simulink model "BLDC_simulator"  (R2024a)
settings: Solver=ode4  StartTime=0.0  StopTime=T  MaxStep=20e-5  RelTol=1e-3  EnableMultiTasking=on
PreLoadFcn:
  | % load scdfocmotorPIDTuning_initial
  | % set_parameters
values from neighbouring files (symbols this model uses):
  current_loop = 1    [BLDC_simulator_init_control.m]    (also in BLDC_simulator_init_control_net_v2_stats_multi.m)
  i_omega = 2.497  * coeff(rand())    [set_parameters_perturbed.m]
  paramPwmCompareAtZeroVolt = 330    [set_parameters_perturbed.m]
  paramPwmCompareMax = 660    [set_parameters_perturbed.m]
  paramPwmComparePerVolt = paramPwmCompareMax/2/BLDC.RatedVoltage    [set_parameters_perturbed.m]
  speed_loop = 1    [BLDC_simulator_init_control.m]    (also in BLDC_simulator_init_control_net_v2_stats_multi.m)
undefined symbols (not defined in the file or in its folder): BLDC, inverter, PID_current, PID_speed, pwm, sampleTime
libraries: nesl_utility x13, fl_lib x12, ee_lib x8, slpidlib x3, simulink x1
(part 1 of 2)
settings Model: ExtModeTrigDuration=8  Creator=The MathWorks, Inc.  LastModifiedBy=39340
settings SolverCC: ZeroCrossAlgorithm=Adaptive  AlgebraicLoopSolver=TrustRegion  MaxZcPerStep=1
settings DataIOCC: InitialState=getstatestruct(op_speedloop)  LimitDataPoints=on  SaveFormat=Structure  InspectSignalLogs=on
settings OptimizationCC: ReuseModelBlockBuffer=off  LifeSpan=Inf
settings DebuggingCC: SolverPrmCheckMsg=warning  InheritedTsInSrcMsg=none  ParameterPrecisionLossMsg=none  UnconnectedInputMsg=warning  UnconnectedOutputMsg=warning  UnconnectedLineMsg=warning  AllowSymbolicDim=off  SFUnexpectedBacktrackingDiag=warning  SFNoUnconditionalDefaultTransitionDiag=warning  SFExecutionAtInitializationDiag=none  ArithmeticOperatorsInVariantConditions=warning
settings HardwareCC: ProdBitPerPointer=32  ProdBitPerSizeT=32  ProdBitPerPtrDiffT=32  ProdLargestAtomicFloat=None  ProdIntDivRoundTo=Undefined  ProdEndianess=Unspecified  ProdWordSize=32  ProdHWDeviceType=ASIC/FPGA->ASIC/FPGA  ProdEqTarget=off
settings ModelReferenceCC: EnableRefExpFcnMdlSchedulingChecks=on  PropagateSignalLabelsOutOfModel=off
settings SFSimCC: SimUseLocalCustomCode=off  CustomCodeUndefinedFunction=UseInterfaceOnly
settings RTWCC: RTWUseLocalCustomCode=off  GPUComputeCapability=3.5  DLArmComputeVersion=19.05
settings CodeAppCC: StateflowObjectComments=on
settings GRTTargetCC: TargetLangStandard=C89/C90 (ANSI)
settings ConfigComp: CovMetricSettings=dw  CovSaveCumulativeToWorkspaceVar=on  CovSaveSingleToWorkspaceVar=on  CovExternalEMLEnable=off  CovSFcnEnable=off
settings SimscapeCC: SimscapeNormalizeSystem=off  SimscapeOperatingPoint=op_innerloop

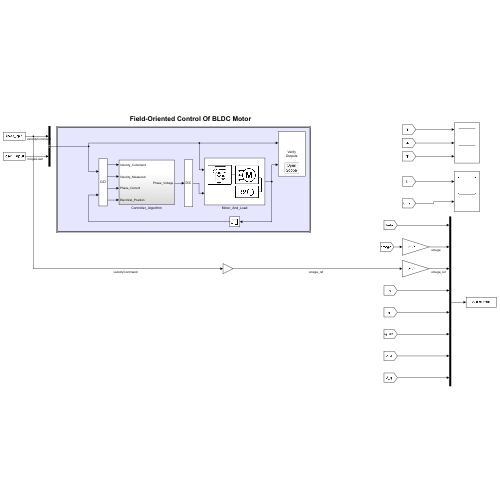
[thumbnail: Simulink's stored preview of the top-level diagram]
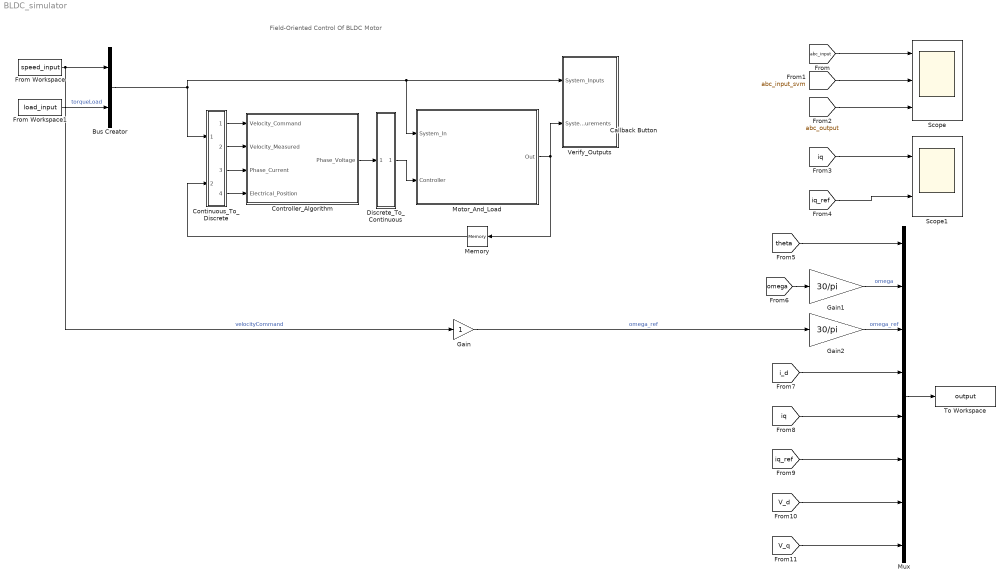
== system BLDC_simulator ==
  note: Field-Oriented Control Of BLDC Motor
  Bus Creator : BusCreator  Inputs=2
  Callback Button : CustomCallbackButton  Configuration="{\"components\":[{\"name\":\"BackgroundImageComponent\",\"settings\":{\"image\":{\"size\":[0,0],\"src\":\"default\",\"srcOrientation\":\"Right\"},\"position\":[0,0,1,1]}},{\"name\":\"ButtonStateComponent\",\"settings\":{\"buttonType\":\"momentary\",\"clickFcn\":\"open_system([bdroot, '\\/Verify_Outputs\\/System_Response']);\\n\",\"onValue\":1,\"position\":[0,0,1,1],\"pressDelay\":\"500\",\"pressFcn\":\"\",\"repeatInterval\":\"0\",\"states\":[{\"horizontalAlignment\":\"center\",\"image\":{\"position\":[0,0,1,1],\"src\":\"default\",\"srcOrientation\":\"Right\"},\"label\":{\"color\":[0.01176470588,0.01176470588,0.01176470588,1],\"icon\":{\"size\":[0,0],\"src\":\"default\",\"srcOrientation\":\"Right\"},\"iconPlacement\":\"left\",\"text\":{\"content\":\"Open Scope\"}},\"labelOffset\":[0,0],\"verticalAlignment\":\"middle\"},{\"horizontalAlignment\":\"center\",\"image\":{\"position\":[0,0,1,1],\"src\":\"default\",\"srcOrientation\":\"Right\"},\"label\":{\"color\":[0.01176470588,0.01176470588,0.01176470588,1],\"icon\":{\"size\":[0,0],\"src\":\"default\",\"srcOrientation\":\"Right\"},\"iconPlacement\":\"left\",\"text\":{\"content\":\"Open Scope\"}},\"labelOffset\":[0,0],\"verticalAlignment\":\"middle\"},{\"horizontalAlignment\":\"center\",\"image\":{\"position\":[0,0,1,1],\"src\":\"default\",\"srcOrientation\":\"Right\"},\"label\":{\"color\":[0.01176470588,0.01176470588,0.01176470588,1],\"icon\":{\"size\":[0,0],\"src\":\"default\",\"srcOrientation\":\"Right\"},\"iconPlacement\":\"left\",\"text\":{\"content\":\"Open Scope\"}},\"labelOffset\":[0,0],\"verticalAlignment\":\"middle\"},{\"horizontalAlignment\":\"center\",\"image\":{\"position\":[0,0,1,1],\"src\":\"default\",\"srcOrientation\":\"Right\"},\"label\":{\"color\":[0.01176470588,0.01176470588,0.01176470588,1],\"icon\":{\"size\":[0,0],\"src\":\"default\",\"srcOrientation\":\"Right\"},\"iconPlacement\":\"left\",\"text\":{\"content\":\"Open Scope\"}},\"labelOffset\":[0,0],\"verticalAlignment\":\"middle\"}]}},{\"name\":\"ForegroundImageComponent\",\"settings\":{\"image\":{\"size\":[0,0],\"src\":\"default\",\"srcOrientation\":\"Right\"},\"isForeground\":1,\"position\":[0,0,1,1]}}],\"settings\":{\"BindingType\":\"standalone\",\"backgroundColor\":[244,244,244,1],\"backgroundOffset\":0.2,\"backgroundOpacity\":1,\"fixedAspectRatio\":\"off\",\"foregroundColor\":[0.01176470588,0.01176470588,0.01176470588,1],\"migratedFromLegacy\":true,\"useBackgroundColor\":true,\"variant\":\"callback\",\"version\":\"R2023a\"},\"type\":\"Button\"}"  CustomBackgroundColor="{\"color\":[0.9568627451,0.9568627451,0.9568627451],\"show\":true}"
  Continuous_To_Discrete : Subsystem
      mask Display: fprintf('C/D')
  Controller_Algorithm : Subsystem
  Discrete_To_Continuous : Subsystem  Description=""
      mask Display: fprintf('D/C')
  From Workspace : FromWorkspace  VariableName=speed_input  SampleTime=-1  OutputAfterFinalValue=Holding final value
  From Workspace1 : FromWorkspace  VariableName=load_input  SampleTime=-1  OutputAfterFinalValue=Holding final value
  Gain : Gain
  Gain1 : Gain  Gain=30/pi
  Gain2 : Gain  Gain=30/pi
  Memory : Memory
  Motor_And_Load : Subsystem
      mask Display: image('focVelocityMotorAndLoadMask.png')
  Mux : Mux  Inputs=8
  Scope : Scope  NumInputPorts=3
  Scope1 : Scope  NumInputPorts=2
  To Workspace : ToWorkspace  VariableName=output  SaveFormat=Structure With Time  SampleTime=-1
      settings: Decimation=1e-2/sampleTime.CurrentControl
  Verify_Outputs : Subsystem  Description=|
      | System Analysis for Speed Control Design
      | 
      | Analyize and plot signals used to analyize performance of
      | speed  control designs
      mask Display: fprintf('Verify\nOutputs')
  wires:
  Discrete_To_Continuous/1(Motor_Commands) -> Motor_And_Load/2(Controller)
  Motor_And_Load/1(Out) -> Memory/1, Verify_Outputs/2(System_Measurements)
  Bus Creator/1 -> Continuous_To_Discrete/1(System_Inputs), Verify_Outputs/1(System_Inputs), Motor_And_Load/1(System_In)
  Continuous_To_Discrete/1(Velocity_Command) -> Controller_Algorithm/1(Velocity_Command)
  Controller_Algorithm/1(Phase_Voltage) -> Discrete_To_Continuous/1(Phase_Voltages)
  Continuous_To_Discrete/3(Phase_Currents) -> Controller_Algorithm/3(Phase_Current)
  Continuous_To_Discrete/4(Electrical_Position) -> Controller_Algorithm/4(Electrical_Position)
  Continuous_To_Discrete/2(Velocity_Measured) -> Controller_Algorithm/2(Velocity_Measured)
  Memory/1 -> Continuous_To_Discrete/2(Motor_Measurements)
  [abc_input] -> Scope/1
  [abc_input_svm] -> Scope/2
  [abc_output] -> Scope/3
  [iq] -> Scope1/1
  [iq_ref] -> Scope1/2
  From Workspace/1 -> Gain/1, Bus Creator/1  "velocityCommand"
  From Workspace1/1 -> Bus Creator/2  "torqueLoad"
  [theta] -> Mux/1
  [omega] -> Gain1/1
  Gain/1 -> Gain2/1  "omega_ref"
  [i_d] -> Mux/4
  [iq] -> Mux/5
  [iq_ref] -> Mux/6
  [V_d] -> Mux/7
  [V_q] -> Mux/8
  Mux/1 -> To Workspace/1
  Gain1/1 -> Mux/2  "omega"
  Gain2/1 -> Mux/3  "omega_ref"

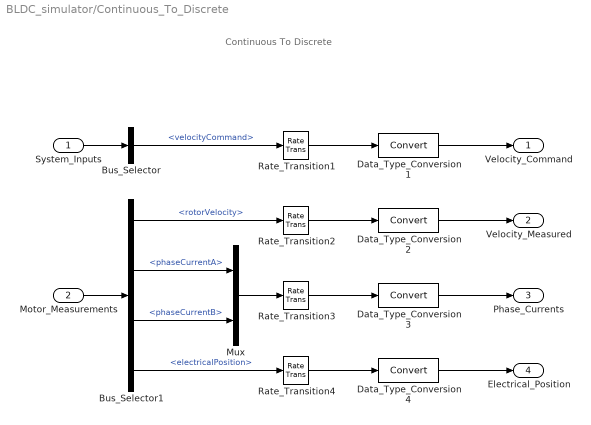
== system BLDC_simulator/Continuous_To_Discrete ==
  note: Continuous To Discrete
  System_Inputs : Inport
  Motor_Measurements : Inport  Port=2
  Bus_Selector : BusSelector  OutputSignals=velocityCommand
  Bus_Selector1 : BusSelector  OutputSignals=motor.rotorVelocity,motor.phaseCurrentA,motor.phaseCurrentB,motor.electricalPosition
  Data_Type_Conversion{1..4} (4 alike) : DataTypeConversion  SaturateOnIntegerOverflow=off  RndMeth=Floor
  Mux : Mux  Inputs=2
  Rate_Transition{1..4} (4 alike) : RateTransition  Integrity=off  Deterministic=off
  Velocity_Command : Outport  VectorParamsAs1DForOutWhenUnconnected=off
  Velocity_Measured : Outport  Port=2  VectorParamsAs1DForOutWhenUnconnected=off
  Phase_Currents : Outport  Port=3  VectorParamsAs1DForOutWhenUnconnected=off
  Electrical_Position : Outport  Port=4  VectorParamsAs1DForOutWhenUnconnected=off
  wires:
  Rate_Transition2/1 -> Data_Type_Conversion2/1
  Data_Type_Conversion2/1 -> Velocity_Measured/1
  Bus_Selector1/1 -> Rate_Transition2/1  "<rotorVelocity>"
  Bus_Selector1/4 -> Rate_Transition4/1  "<electricalPosition>"
  Mux/1 -> Rate_Transition3/1
  Bus_Selector1/3 -> Mux/2  "<phaseCurrentB>"
  Bus_Selector1/2 -> Mux/1  "<phaseCurrentA>"
  Data_Type_Conversion3/1 -> Phase_Currents/1
  Rate_Transition3/1 -> Data_Type_Conversion3/1
  Rate_Transition4/1 -> Data_Type_Conversion4/1
  Data_Type_Conversion4/1 -> Electrical_Position/1
  Motor_Measurements/1 -> Bus_Selector1/1
  Data_Type_Conversion1/1 -> Velocity_Command/1
  Rate_Transition1/1 -> Data_Type_Conversion1/1
  Bus_Selector/1 -> Rate_Transition1/1  "<velocityCommand>"
  System_Inputs/1 -> Bus_Selector/1

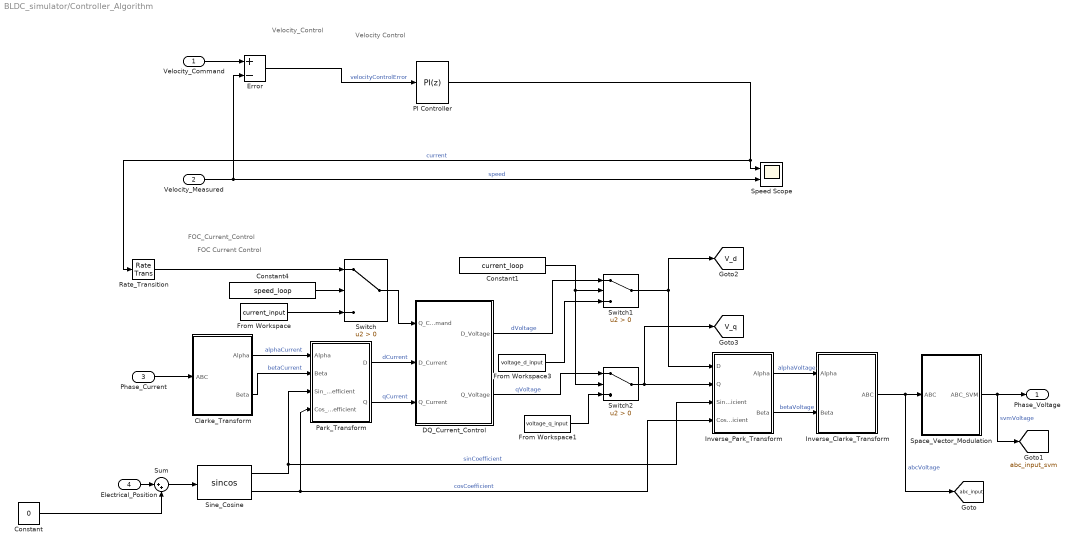
== system BLDC_simulator/Controller_Algorithm ==
  note: Velocity Control
  note: FOC_Current_Control
  note: Velocity_Control
  note: FOC Current Control
  Velocity_Command : Inport  OutDataTypeStr=single  SampleTime=sampleTime.VelocityControl
  Velocity_Measured : Inport  Port=2  OutDataTypeStr=single  SampleTime=sampleTime.VelocityControl
  Phase_Current : Inport  Port=3  OutDataTypeStr=single  SampleTime=sampleTime.CurrentControl
  Electrical_Position : Inport  Port=4  OutDataTypeStr=single  SampleTime=sampleTime.CurrentControl
  Clarke_Transform : Subsystem
      mask Display:
      | port_label('input',1,'ABC')
      | port_label('output',1,'\alpha','texmode', 'on')
      | port_label('output',2,'\beta','texmode', 'on')
  Constant : Constant  Value=0
  Constant1 : Constant  Value=current_loop
  Constant4 : Constant  Value=speed_loop
  DQ_Current_Control : Subsystem
  Error : Sum  Inputs=+-
  From Workspace : FromWorkspace  VariableName=current_input  SampleTime=-1
  From Workspace1 : FromWorkspace  VariableName=voltage_q_input  SampleTime=-1
  From Workspace3 : FromWorkspace  VariableName=voltage_d_input  SampleTime=-1
  Inverse_Clarke_Transform : Subsystem  VariantControl=INVERSE_CLARKE_TRANSFORM
      mask Display:
      | port_label('input',1,'\alpha','texmode', 'on')
      | port_label('input',2,'\beta','texmode', 'on')
      | port_label('output',1,'ABC')
  Inverse_Park_Transform : Subsystem
      mask Display:
      | port_label('input',1,'D')
      | port_label('input',2,'Q')
      | port_label('input',3,'Sin')
      | port_label('input',4,'Cos')
      | port_label('output',1,'\alpha','texmode', 'on')
      | port_label('output',2,'\beta','texmode', 'on')
  PI Controller : slpidlib/PID Controller  Controller=PI  Form=Parallel  TimeDomain=Discrete-time  UseExternalTs=off  SampleTime=sampleTime.VelocityControl  IntegratorMethod=Forward Euler  FilterMethod=Forward Euler  ControllerParametersSource=internal  P=PID_speed.p  I=PID_speed.i  UseKiTs=off  D=5e-5  UseExternalDerivativeSource=off  N=20000  UseFilter=off  TunerSelectOption=Transfer Function Based (PID Tuner App)  InitialConditionSource=internal  InitialConditionForIntegrator=0  InitialConditionForFilter=0  DifferentiatorICPrevScaledInput=0  ExternalReset=none  TrackingMode=off  Kt=1  LimitOutput=on  SatLimitsSource=internal  UpperSaturationLimit=BLDC.CurrentMax  LowerSaturationLimit=-BLDC.CurrentMax  LinearizeAsGain=off  AntiWindupMode=clamping  Kb=1000  LimitIntegrator=off  UpperIntegratorSaturationLimit=inf  LowerIntegratorSaturationLimit=-inf  POutMin=[]  POutMax=[]  IOutMin=[]  IOutMax=[]  DOutMin=[]  DOutMax=[]  NOutMin=[]  NOutMax=[]  SumOutMin=[]  SumOutMax=[]  SaturationOutMin=[]  SaturationOutMax=[]  PParamMin=[]  PParamMax=[]  IParamMin=[]  IParamMax=[]  DParamMin=[]  DParamMax=[]  NParamMin=[]  NParamMax=[]  KbParamMin=[]  KbParamMax=[]  KtParamMin=[]  KtParamMax=[]  KbOutMin=[]  KbOutMax=[]  KtOutMin=[]  KtOutMax=[]  IntegratorOutMin=[]  IntegratorOutMax=[]  FilterOutMin=[]  FilterOutMax=[]  SumI1OutMin=[]  SumI1OutMax=[]  SumI2OutMin=[]  SumI2OutMax=[]  SumI3OutMin=[]  SumI3OutMax=[]  SumI4OutMin=[]  SumI4OutMax=[]  SumDOutMin=[]  SumDOutMax=[]  DifferentiatorOutMin=[]  DifferentiatorOutMax=[]  FilterDiffOutCoefMin=[]  FilterDiffOutCoefMax=[]  ReciprocalOutMin=[]  ReciprocalOutMax=[]  SumDenOutMin=[]  SumDenOutMax=[]  SumNumOutMin=[]  SumNumOutMax=[]  DivideOutMin=[]  DivideOutMax=[]  UdiffTsProdOutMin=[]  UdiffTsProdOutMax=[]  NTsProdOutMin=[]  NTsProdOutMax=[]  UintegralTsProdOutMin=[]  UintegralTsProdOutMax=[]  UngainTsProdOutMin=[]  UngainTsProdOutMax=[]  ClampingZeroOutDataTypeStr=Inherit: Inherit via back propagation  ClampingZeroOutMin=[]  ClampingZeroOutMax=[]  FilterDenConstantOutDataTypeStr=Inherit: Inherit via back propagation  FilterDenConstantOutMin=[]  FilterDenConstantOutMax=[]  PCopyOutDataTypeStr=Inherit: Inherit via back propagation  PCopyOutMin=[]  PCopyOutMax=[]  NCopyOutDataTypeStr=Inherit: Inherit via back propagation  NCopyOutMin=[]  NCopyOutMax=[]  IntegratorContinuousStateAttributes=''  IntegratorStateMustResolveToSignalObject=off  IntegratorRTWStateStorageClass=Auto  FilterContinuousStateAttributes=''  FilterStateMustResolveToSignalObject=off  FilterRTWStateStorageClass=Auto  ParallelPVariant=InternalParameters  IdealPVariant=Disabled  IVariant=InternalParameters  DVariant=Disabled  IntegratorVariant=Discrete  SatVariant=Enabled  AWVariant=DiscClampingParallel  PCopyVariant=Disabled  TRVariant=Disabled  FdbkBlocksVariant=Forward  IdealPFdbkVariant=Disabled  SatFdbkVariant=Disabled  DerivativeFilterVariant=Disabled  NVariant=Disabled  NCopyVariant=Disabled_SignalSpec  FilterICVariant=Disabled  IntegratorICVariant=InternalICs  ExternalResetVariant=Disabled  TRSumVariant=Passthrough  SumFdbkVariant=Disabled  SumVariant=Sum_PI  TsampFilterVariant=InternalTs  TsampNgainVariant=Passthrough  TsampIntegralVariant=Disabled_SignalSpec  ExternalSaturationOutDataTypeStr=Inherit: Same as second input  DerivativeSourceVariant=Disabled
  Park_Transform : Subsystem
      mask Display:
      | port_label('input',1,'\alpha','texmode', 'on')
      | port_label('input',2,'\beta','texmode', 'on')
      | port_label('input',3,'Sin')
      | port_label('input',4,'Cos')
      | port_label('output',1,'D')
      | port_label('output',2,'Q')
  Rate_Transition : RateTransition  Integrity=off
  Sine_Cosine : Trigonometry  Operator=sincos
  Space_Vector_Modulation : Subsystem  VariantControl=SpaceVectorModulation_JB
      mask Display:
      | plot([0.000 0.020 0.041 0.061 0.082 0.102 0.122 0.143 0.163 0.184 0.204 0.224 0.245 0.265 0.286 0.306 0.327 0.347 0.367 0.388 0.408 0.429 0.449 0.469 0.490 0.510 0.531 0.551 0.571 0.592 0.612 0.633 0.653 0.673 0.694 0.714 0.735 0.755 0.776 0.796 0.816 0.837 0.857 0.878 0.898 0.918 0.939 0.959 0.980 1.000 ], ...
      |      [0.500 0.586 0.671 0.753 0.831 0.858 0.875 0.885 0.890 0.887 0.879 0.864 0.844 0.855 0.872 0.884 0.889 0.888 0.881 0.867 0.847 0.793 0.713 0.629 0.543 0.457 0.371 0.287 0.207 0.153 0.133 0.119 0.112 0.111 0.116 0.128 0.145 0.156 0.136 0.121 0.113 0.110 0.115 0.125 0.142 0.169 0.247 0.329 0.414 0.500 ])
  Speed Scope : Scope  NumInputPorts=2
  Sum : Sum  Inputs=|++
  Switch : Switch  Criteria=u2 > Threshold  SaturateOnIntegerOverflow=off  InputSameDT=off
  Switch1 : Switch  Criteria=u2 > Threshold  SaturateOnIntegerOverflow=off  InputSameDT=off
  Switch2 : Switch  Criteria=u2 > Threshold  SaturateOnIntegerOverflow=off  InputSameDT=off
  Phase_Voltage : Outport  VectorParamsAs1DForOutWhenUnconnected=off
  tag scope: V_d=global, V_q=global, abc_input=global, abc_input_svm=global
  wires:
  Inverse_Park_Transform/2(Beta) -> Inverse_Clarke_Transform/2(Beta)  "betaVoltage"
  Error/1 -> PI Controller/1  "velocityControlError"
  Sine_Cosine/1 -> Park_Transform/3(Sin_Coefficient), Inverse_Park_Transform/3(Sin_Coefficient)  "sinCoefficient"
  Inverse_Clarke_Transform/1(ABC) -> Space_Vector_Modulation/1(ABC), [abc_input]  "abcVoltage"
  Inverse_Park_Transform/1(Alpha) -> Inverse_Clarke_Transform/1(Alpha)  "alphaVoltage"
  Phase_Current/1 -> Clarke_Transform/1(ABC)
  Park_Transform/1(D) -> DQ_Current_Control/2(D_Current)  "dCurrent"
  Sine_Cosine/2 -> Park_Transform/4(Cos_Coefficient), Inverse_Park_Transform/4(Cos_Coefficient)  "cosCoefficient"
  Velocity_Command/1 -> Error/1
  Clarke_Transform/1(Alpha) -> Park_Transform/1(Alpha)  "alphaCurrent"
  PI Controller/1 -> Speed Scope/1, Rate_Transition/1  "current"
  Clarke_Transform/2(Beta) -> Park_Transform/2(Beta)  "betaCurrent"
  Space_Vector_Modulation/1(ABC_SVM) -> Phase_Voltage/1, [abc_input_svm]  "svmVoltage"
  Park_Transform/2(Q) -> DQ_Current_Control/3(Q_Current)  "qCurrent"
  Velocity_Measured/1 -> Speed Scope/2, Error/2  "speed"
  Switch1/1 -> Inverse_Park_Transform/1(D), [V_d]
  From Workspace3/1 -> Switch1/3
  DQ_Current_Control/1(D_Voltage) -> Switch1/1  "dVoltage"
  Switch2/1 -> [V_q], Inverse_Park_Transform/2(Q)
  From Workspace1/1 -> Switch2/3
  DQ_Current_Control/2(Q_Voltage) -> Switch2/1  "qVoltage"
  Switch/1 -> DQ_Current_Control/1(Q_Command)
  Rate_Transition/1 -> Switch/1
  Constant4/1 -> Switch/2
  Constant1/1 -> Switch2/2, Switch1/2
  From Workspace/1 -> Switch/3
  Electrical_Position/1 -> Sum/1
  Constant/1 -> Sum/2
  Sum/1 -> Sine_Cosine/1

== system BLDC_simulator/Discrete_To_Continuous ==
  note: Discrete To Continuous
  Phase_Voltages : Inport
  Bus_Creator1 : BusCreator  Inputs=1
  Data_Type_Conversion : DataTypeConversion  SaturateOnIntegerOverflow=off  RndMeth=Floor
  Rate_Transition : RateTransition  Integrity=off  Deterministic=off
  Motor_Commands : Outport  VectorParamsAs1DForOutWhenUnconnected=off
  wires:
  Rate_Transition/1 -> Bus_Creator1/1  "phaseVoltages"
  Data_Type_Conversion/1 -> Rate_Transition/1
  Phase_Voltages/1 -> Data_Type_Conversion/1
  Bus_Creator1/1 -> Motor_Commands/1

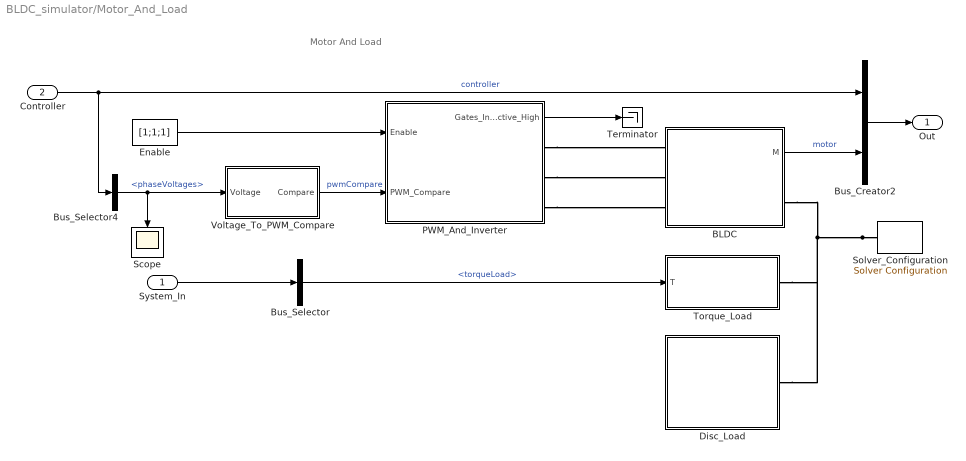
== system BLDC_simulator/Motor_And_Load ==
  note: Motor And Load
  System_In : Inport
  Controller : Inport  Port=2
  BLDC : Subsystem
      mask Display:
      | image('pmsmMask.png')
      | text(0.03, 0.80, 'A', 'HorizontalAlignment', 'Left')
      | text(0.03, 0.50, 'B', 'HorizontalAlignment', 'Left')
      | text(0.03, 0.20, 'C', 'HorizontalAlignment', 'Left')
      | text(0.98, 0.75, 'M', 'HorizontalAlignment', 'Right')
      | text(0.98, 0.25, 'R', 'HorizontalAlignment', 'Right')
  Bus_Creator2 : BusCreator  Inputs=2
  Bus_Selector : BusSelector  OutputSignals=torqueLoad
  Bus_Selector4 : BusSelector  OutputSignals=phaseVoltages
  Disc_Load : Subsystem  VariantControl=loadType == motorLoad.disc
      mask Display: image('discAluminumMask.png')
  Enable : Constant  Value=[1;1;1]
  PWM_And_Inverter : Subsystem  VariantControl=variantPwm == enumPwm.behavior
      mask Display:
      | image('pwmAndInverterMask.png')
      | port_label('input',1,'En')
      | port_label('input',2,'Compare')
      | text(0.98, 0.88, 'G', 'HorizontalAlignment', 'Right')
      | text(0.98, 0.62, 'A', 'HorizontalAlignment', 'Right')
      | text(0.98, 0.38, 'B', 'HorizontalAlignment', 'Right')
      | text(0.98, 0.12, 'C', 'HorizontalAlignment', 'Right')
  Scope : Scope
  Solver_Configuration : nesl_utility/Solver Configuration  PhysicalDomain=network_engine_domain  SubClassName=solver  LeftPortType=input  RightPortType=generic  Tones=[]  Harmonics=[]  SimulateNoise=off  Profile=off  UseLocalSampling=off  EnableSwitchedLinearOptims=on  FrequencyDomain=off  UseCCode=off  RelTol=0.001  AbsTol=1e-06  MinStep=1e-09  ToWorkspace=off  RevertToSquareIcSolve=off  NumHomotopyIterations=100  PhasorMode=off  PhasorModeNumHarmonics=1  ConsistencySolver=NEWTON_FTOL  IndexReductionMethod=DerivativeReplacement  DoDC=off  ResidualTolerance=1e-9  ConsistencyTolSource=GLOBAL  ConsistencyAbsTol=0.001  ConsistencyRelTol=0.001  ConsistencyTolFactor=0.001  UseLocalSolver=on  LocalSolverChoice=NE_BACKWARD_EULER_ADVANCER  ResolveIndetEquations=on  FunctionEvalNumThread=1  LocalSolverSampleTime=sampleTime.CurrentControl  DoFixedCost=on  MaxNonlinIter=3  MaxModeIter=2  ComputeImpulses=off  ImpulseIterations=2  LinearAlgebra=Sparse  LinearAlgebraNumThread=0  EquationFormulation=NE_TIME_EF  DelaysMemoryBudget=1024  AutomaticFiltering=on  FilteringTimeConstant=0.001  PartitionStorageMethod=AS_NEEDED  PartitionMemoryBudget=1024  PartitionMethod=FAST  MultibodyUseLocalSolver=off  MultibodyLocalSolverChoice=ODE1  MultibodyLocalSolverSampleTime=0.001
  Terminator : Terminator
  Torque_Load : Subsystem  VariantControl=loadType == motorLoad.disc
      mask Display:
      | image('torqueLoadMask.png')
      | text(0.03, 0.5, 'T', 'HorizontalAlignment', 'Left')
      | text(0.98, 0.5, 'R', 'HorizontalAlignment', 'Right')
  Voltage_To_PWM_Compare : Subsystem
  Out : Outport  VectorParamsAs1DForOutWhenUnconnected=off
  wires:
  Enable/1 -> PWM_And_Inverter/1(Enable)
  Bus_Selector4/1 -> Scope/1, Voltage_To_PWM_Compare/1(Voltage)  "<phaseVoltages>"
  Bus_Selector/1 -> Torque_Load/1(T)  "<torqueLoad>"
  System_In/1 -> Bus_Selector/1
  BLDC/1(M) -> Bus_Creator2/2  "motor"
  Bus_Creator2/1 -> Out/1
  Controller/1 -> Bus_Creator2/1, Bus_Selector4/1  "controller"
  Voltage_To_PWM_Compare/1(Compare) -> PWM_And_Inverter/2(PWM_Compare)  "pwmCompare"
  PWM_And_Inverter/1(Gates_Individual_Active_High) -> Terminator/1
  connections:
  Solver_Configuration/RConn1 -- Disc_Load/RConn1 -- Torque_Load/RConn1 -- BLDC/RConn1
  PWM_And_Inverter/RConn2 -- BLDC/LConn2
  PWM_And_Inverter/RConn3 -- BLDC/LConn3
  PWM_And_Inverter/RConn1 -- BLDC/LConn1

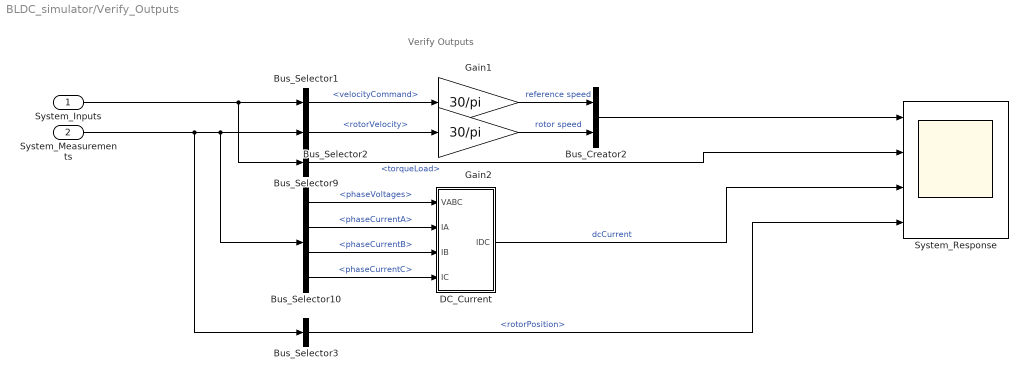
== system BLDC_simulator/Verify_Outputs ==
  note: Verify Outputs
  System_Inputs : Inport
  System_Measurements : Inport  Port=2
  Bus_Creator2 : BusCreator  Inputs=2
  Bus_Selector1 : BusSelector  OutputSignals=velocityCommand
  Bus_Selector10 : BusSelector  OutputSignals=controller.phaseVoltages,motor.phaseCurrentA,motor.phaseCurrentB,motor.phaseCurrentC
  Bus_Selector2 : BusSelector  OutputSignals=motor.rotorVelocity
  Bus_Selector3 : BusSelector  OutputSignals=motor.rotorPosition
  Bus_Selector9 : BusSelector  OutputSignals=torqueLoad
  DC_Current : Subsystem
  Gain1 : Gain  Gain=30/pi
  Gain2 : Gain  Gain=30/pi
  System_Response : Scope  NumInputPorts=4
  wires:
  DC_Current/1(IDC) -> System_Response/3  "dcCurrent"
  Bus_Selector10/1 -> DC_Current/1(VABC)  "<phaseVoltages>"
  Bus_Selector10/4 -> DC_Current/4(IC)  "<phaseCurrentC>"
  Bus_Selector10/3 -> DC_Current/3(IB)  "<phaseCurrentB>"
  Bus_Selector10/2 -> DC_Current/2(IA)  "<phaseCurrentA>"
  Bus_Selector9/1 -> System_Response/2  "<torqueLoad>"
  Bus_Selector2/1 -> Gain2/1  "<rotorVelocity>"
  Bus_Selector1/1 -> Gain1/1  "<velocityCommand>"
  System_Measurements/1 -> Bus_Selector3/1, Bus_Selector10/1, Bus_Selector2/1
  System_Inputs/1 -> Bus_Selector1/1, Bus_Selector9/1
  Bus_Selector3/1 -> System_Response/4  "<rotorPosition>"
  Bus_Creator2/1 -> System_Response/1
  Gain1/1 -> Bus_Creator2/1  "reference speed"
  Gain2/1 -> Bus_Creator2/2  "rotor speed"

== system BLDC_simulator/Controller_Algorithm/Clarke_Transform ==
  note: Clarke Transform
  note: Converts balanced three-phase quantities into balanced two-phase quantities.
      | The A and B phases are converted to the direct axis (alpha) component and the quadrature axis (beta) component.
      | The alpha and beta components are still dependent on time and speed.
  ABC : Inport
  A : Selector  IndexMode=Zero-based  InputPortWidth=2  IndexOptions=Index vector (dialog)  Indices=0  OutputSizes=1
  Add : Sum  OutDataTypeStr=Inherit: Same as first input
  Alpha_Gain : Gain  Gain=1/sqrt(3)
  B : Selector  IndexMode=Zero-based  InputPortWidth=2  IndexOptions=Index vector (dialog)  Indices=1  OutputSizes=1
  Beta_Gain : Gain  Gain=2/sqrt(3)
  Alpha : Outport  VectorParamsAs1DForOutWhenUnconnected=off
  Beta : Outport  Port=2  VectorParamsAs1DForOutWhenUnconnected=off
  wires:
  Add/1 -> Beta/1
  B/1 -> Beta_Gain/1
  Beta_Gain/1 -> Add/2
  ABC/1 -> A/1, B/1
  Alpha_Gain/1 -> Add/1
  A/1 -> Alpha_Gain/1, Alpha/1

== system BLDC_simulator/Controller_Algorithm/DQ_Current_Control ==
  note: DQ Current Control
  Q_Command : Inport  SampleTime=sampleTime.CurrentControl
  D_Current : Inport  Port=2
  Q_Current : Inport  Port=3
  D_Command : Constant  Value=0  OutDataTypeStr=single  SampleTime=-1
  D_Current_Control : Subsystem
  Q_Current_Control : Subsystem
  D_Voltage : Outport  VectorParamsAs1DForOutWhenUnconnected=off
  Q_Voltage : Outport  Port=2  VectorParamsAs1DForOutWhenUnconnected=off
  tag scope: iq=global, iq_ref=global
  wires:
  Q_Current_Control/1(Voltage) -> Q_Voltage/1  "VQ"
  D_Current_Control/1(Voltage) -> D_Voltage/1  "VD"
  D_Command/1 -> D_Current_Control/1(Current_Command)  "IDcmd"
  Q_Command/1 -> [iq_ref], Q_Current_Control/1(Current_Command)  "IQcmd"
  Q_Current/1 -> [iq], Q_Current_Control/2(Current_Measured)  "IQmea"
  D_Current/1 -> D_Current_Control/2(Current_Measured)  "IDmea"

== system BLDC_simulator/Controller_Algorithm/Inverse_Clarke_Transform ==
  note: Inverse Clarke Transform
  note: Converts direct axis (alpha) component and the quadrature axis (beta) component to balanced three-phase quantities
      | The alpha and beta components are dependent on time and speed.
  Alpha : Inport
  Beta : Inport  Port=2
  Add : Sum  Inputs=-+  OutDataTypeStr=Inherit: Same as first input
  Add1 : Sum  Inputs=--  OutDataTypeStr=Inherit: Same as first input
  Gain : Gain  Gain=1/2
  Gain1 : Gain  Gain=sqrt(3)/2
  Mux : Mux  Inputs=3
  ABC : Outport  VectorParamsAs1DForOutWhenUnconnected=off
  wires:
  Gain/1 -> Add1/1, Add/1
  Gain1/1 -> Add1/2, Add/2
  Add/1 -> Mux/2
  Add1/1 -> Mux/3
  Beta/1 -> Gain1/1
  Alpha/1 -> Mux/1, Gain/1
  Mux/1 -> ABC/1

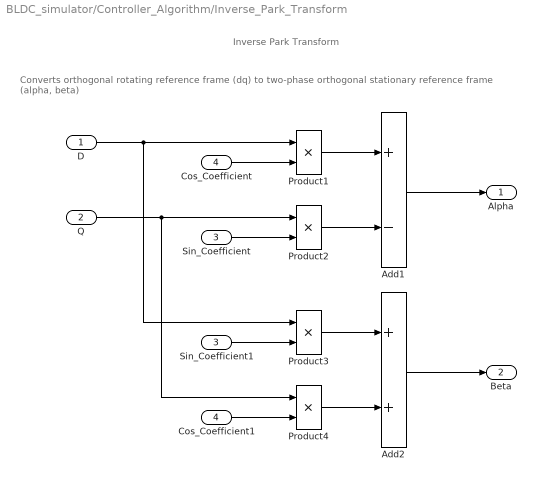
== system BLDC_simulator/Controller_Algorithm/Inverse_Park_Transform ==
  note: Inverse Park Transform
  note: Converts orthogonal rotating reference frame (dq) to two-phase orthogonal stationary reference frame (alpha, beta)
  D : Inport
  Q : Inport  Port=2
  Sin_Coefficient : Inport  Port=3
  Cos_Coefficient : Inport  Port=4
  Add1 : Sum  Inputs=+-  OutDataTypeStr=Inherit: Same as first input
  Add2 : Sum  OutDataTypeStr=Inherit: Same as first input
  Cos_Coefficient1 : InportShadow  Port=4
  Product{1..4} (4 alike) : Product  RndMeth=Simplest
  Sin_Coefficient1 : InportShadow  Port=3
  Alpha : Outport  VectorParamsAs1DForOutWhenUnconnected=off
  Beta : Outport  Port=2  VectorParamsAs1DForOutWhenUnconnected=off
  wires:
  Add2/1 -> Beta/1
  Add1/1 -> Alpha/1
  Product3/1 -> Add2/1
  Product4/1 -> Add2/2
  Product1/1 -> Add1/1
  Product2/1 -> Add1/2
  Cos_Coefficient1/1 -> Product4/2
  Sin_Coefficient/1 -> Product2/2
  D/1 -> Product3/1, Product1/1
  Q/1 -> Product2/1, Product4/1
  Sin_Coefficient1/1 -> Product3/2
  Cos_Coefficient/1 -> Product1/2

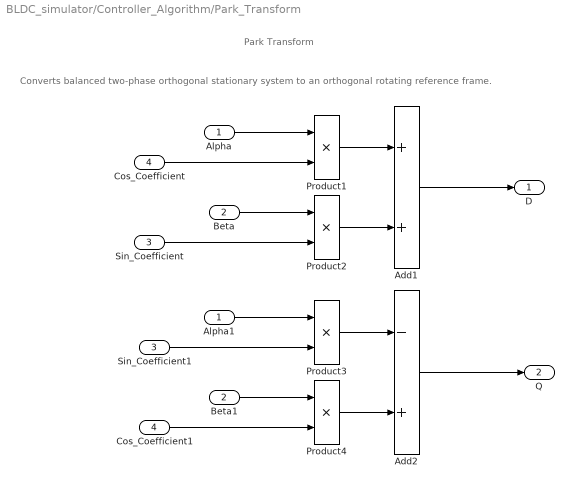
== system BLDC_simulator/Controller_Algorithm/Park_Transform ==
  note: Park Transform
  note: Converts balanced two-phase orthogonal stationary system to an orthogonal rotating reference frame.
  Alpha : Inport
  Beta : Inport  Port=2
  Sin_Coefficient : Inport  Port=3
  Cos_Coefficient : Inport  Port=4
  Add1 : Sum  OutDataTypeStr=Inherit: Same as first input
  Add2 : Sum  Inputs=-+  OutDataTypeStr=Inherit: Same as first input
  Alpha1 : InportShadow
  Beta1 : InportShadow  Port=2
  Cos_Coefficient1 : InportShadow  Port=4
  Product{1..4} (4 alike) : Product  RndMeth=Simplest
  Sin_Coefficient1 : InportShadow  Port=3
  D : Outport  VectorParamsAs1DForOutWhenUnconnected=off
  Q : Outport  Port=2  VectorParamsAs1DForOutWhenUnconnected=off
  wires:
  Product3/1 -> Add2/1
  Product4/1 -> Add2/2
  Product1/1 -> Add1/1
  Product2/1 -> Add1/2
  Alpha1/1 -> Product3/1
  Sin_Coefficient1/1 -> Product3/2
  Cos_Coefficient1/1 -> Product4/2
  Beta1/1 -> Product4/1
  Alpha/1 -> Product1/1
  Cos_Coefficient/1 -> Product1/2
  Beta/1 -> Product2/1
  Sin_Coefficient/1 -> Product2/2
  Add1/1 -> D/1
  Add2/1 -> Q/1

== system BLDC_simulator/Controller_Algorithm/Space_Vector_Modulation ==
  note: Space Vector Modulation
  ABC : Inport
  Add : Sum
  Add1 : Sum  Inputs=+-
  Gain : Gain  Gain=0.5  OutDataTypeStr=Inherit: Same as input
  Max : MinMax  Function=max
  Min : MinMax
  ABC_SVM : Outport  VectorParamsAs1DForOutWhenUnconnected=off
  wires:
  Add/1 -> Gain/1
  Max/1 -> Add/1
  Min/1 -> Add/2
  Gain/1 -> Add1/2
  ABC/1 -> Add1/1, Max/1, Min/1
  Add1/1 -> ABC_SVM/1

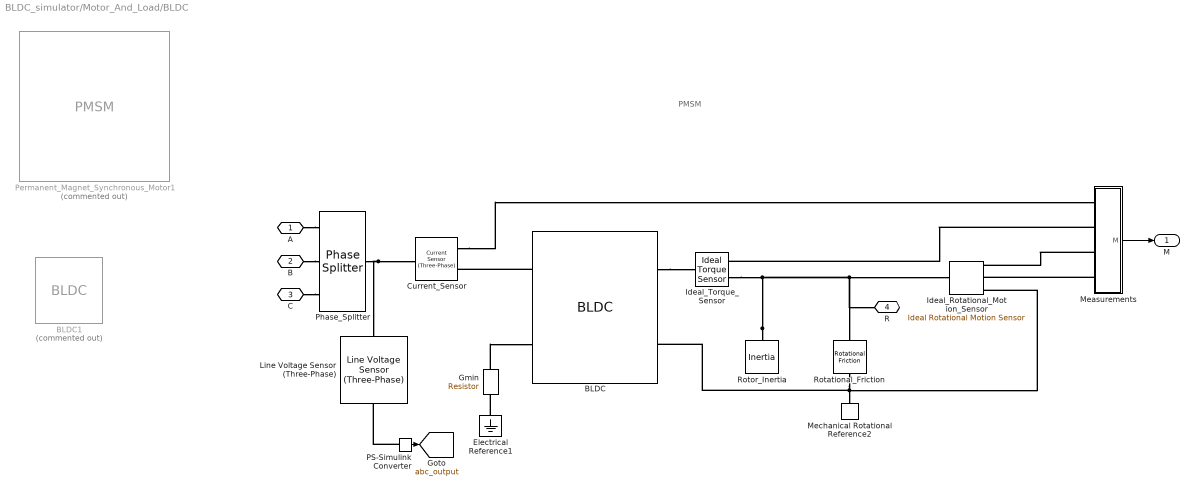
== system BLDC_simulator/Motor_And_Load/BLDC ==
  note: PMSM
  BLDC : ee_lib/Electromechanical/Permanent Magnet/BLDC  Tag={'toolbox/physmod/elec/library/m/ee_lib_parts';'Electromechanical/Permanent_Magnet/BLDC/Maxon/ECXTORQUE_22XL_48.xml'}  port_option=ee.enum.threePhasePort.composite  rotor_param=ee.enum.pmsm.backemf.trapezoidflux  pm_flux_linkage=BLDC.FluxLinkage Wb  theta_constant="31.25*4/BLDC.PolePairs  deg"  emf_max=9.6 % Parameter not set V  w_meas=600 % Parameter not set rpm  DphiDtheta_tab=[0, -.1528, -.1528, .1528, .1528, 0] % Parameter not set Wb/rad  back_emf_tab=[0, -9.6, -9.6, 9.6, 9.6, 0] % Parameter not set V  rotor_angle_tab=[0, 7.5, 22.5, 37.5, 52.5, 60] % Parameter not set deg  nPolePairs=BLDC.PolePairs  axes_param=ee.enum.rotorangle.daxis  winding_type=ee.enum.statorconnection.wye  stator_param=ee.enum.statorparam.LdLqL0  machine_param=ee.enum.dqparameterization.constant  Ld=BLDC.InductanceLd H  Lq=BLDC.InductanceLq H  idVec=[-200, 0, 200] % Parameter not set A  iqVec=[-200, 0, 200] % Parameter not set A  LdMatrix=0.00022 * ones(3, 3) % Parameter not set H  LqMatrix=0.00022 * ones(3, 3) % Parameter not set H  L0="BLDC.InductanceL0  % Assumed inductance value H"  Ls=Ls % Parameter not set H  Lm=0 % Parameter not set H  Ms=Ms % Parameter not set H  Rs=BLDC.StatorPhaseResistance Ohm  zero_sequence=ee.enum.park.zerosequence.include  loss_param=ee.enum.ironloss.none  losses_oc=[0, 0, 0] % Parameter not set W  losses_sc=[0, 0, 0] % Parameter not set W  f_losses=60 % Parameter not set Hz  Isc_losses=95 % Parameter not set A  J=0 kg*m^2  lam=0 % Parameter not set N*m/(rad/s)  i_d_specify=off  i_d_priority=None  i_d=0 A  i_d_nominal_specify=off  i_d_nominal_value=1  i_d_nominal_unit=A  i_q_specify=off  i_q_priority=None  i_q=0 A  i_q_nominal_specify=off  i_q_nominal_value=1  i_q_nominal_unit=A  torque_specify=off  torque_priority=None  torque=0 N*m  torque_nominal_specify=off  torque_nominal_value=1  torque_nominal_unit=N*m  angular_velocity_specify=on  angular_velocity_priority=Low  angular_velocity=BLDC.RotorVelocityInit rpm  angular_velocity_nominal_specify=off  angular_velocity_nominal_value=1  angular_velocity_nominal_unit=rpm  angular_position_specify=off  angular_position_priority=High  angular_position=0 deg  angular_position_nominal_specify=off  angular_position_nominal_value=1  angular_position_nominal_unit=deg  alpha=0.00393 % Parameter not set 1/K  alpha_flux=-0.001 % Parameter not set 1/K  Tmeas=298.15 % Parameter not set K  stator_thermal_mass=100 % Parameter not set J/K  rotor_thermal_mass=200 % Parameter not set J/K  Rm_percent_rotor=90  Rd_percent_rotor=30  temperatureA_specify=off  temperatureA_priority=High  temperatureA=25 degC  temperatureA_nominal_specify=off  temperatureA_nominal_value=1  temperatureA_nominal_unit=degC  temperatureB_specify=off  temperatureB_priority=High  temperatureB=25 degC  temperatureB_nominal_specify=off  temperatureB_nominal_value=1  temperatureB_nominal_unit=degC  temperatureC_specify=off  temperatureC_priority=High  temperatureC=25 degC  temperatureC_nominal_specify=off  temperatureC_nominal_value=1  temperatureC_nominal_unit=degC  temperatureR_specify=off  temperatureR_priority=High  temperatureR=25 degC  temperatureR_nominal_specify=off  temperatureR_nominal_value=1  temperatureR_nominal_unit=degC
      settings: AttributesFormatString=Maxon:ECXTORQUE_22XL_48  InternalSimscapePortConfiguration="{\"Bottom\":[],\"Left\":[{\"id\":\"N\",\"label\":\"~\",\"type\":\"foundation.electrical.three_phase\"},{\"id\":\"n\",\"label\":\"n\",\"type\":\"foundation.electrical.electrical\"}],\"Right\":[{\"id\":\"R\",\"label\":\"R\",\"type\":\"foundation.mechanical.rotational.rotational\"},{\"id\":\"C\",\"label\":\"C\",\"type\":\"foundation.mechanical.rotational.rotational\"}],\"Top\":[]}"
  BLDC1 : ee_lib/Electromechanical/Permanent Magnet/BLDC  Tag={'toolbox/physmod/elec/library/m/ee_lib_parts';'Electromechanical/Permanent_Magnet/BLDC/Maxon/ECXTORQUE_22XL_48.xml'}  Commented=on  port_option=ee.enum.threePhasePort.composite  rotor_param=ee.enum.pmsm.backemf.trapezoidflux  pm_flux_linkage=0.0119333333333333 Wb  theta_constant=31.25 % Assumed angle deg  emf_max=9.6 % Parameter not set V  w_meas=600 % Parameter not set rpm  DphiDtheta_tab=[0, -.1528, -.1528, .1528, .1528, 0] % Parameter not set Wb/rad  back_emf_tab=[0, -9.6, -9.6, 9.6, 9.6, 0] % Parameter not set V  rotor_angle_tab=[0, 7.5, 22.5, 37.5, 52.5, 60] % Parameter not set deg  nPolePairs=4  axes_param=ee.enum.rotorangle.daxis  winding_type=ee.enum.statorconnection.wye  stator_param=ee.enum.statorparam.LdLqL0  machine_param=ee.enum.dqparameterization.constant  Ld=1.44 mH  Lq=1.44 mH  idVec=[-200, 0, 200] % Parameter not set A  iqVec=[-200, 0, 200] % Parameter not set A  LdMatrix=0.00022 * ones(3, 3) % Parameter not set H  LqMatrix=0.00022 * ones(3, 3) % Parameter not set H  L0="1.44  % Assumed inductance value mH"  Ls=Ls % Parameter not set H  Lm=0 % Parameter not set H  Ms=Ms % Parameter not set H  Rs=2.065 Ohm  zero_sequence=ee.enum.park.zerosequence.exclude  loss_param=ee.enum.ironloss.none  losses_oc=[0, 0, 0] % Parameter not set W  losses_sc=[0, 0, 0] % Parameter not set W  f_losses=60 % Parameter not set Hz  Isc_losses=95 % Parameter not set A  J=4.97e-07 kg*m^2  lam=0 % Parameter not set N*m/(rad/s)  i_d_specify=off  i_d_priority=None  i_d=0 A  i_d_nominal_specify=off  i_d_nominal_value=1  i_d_nominal_unit=A  i_q_specify=off  i_q_priority=None  i_q=0 A  i_q_nominal_specify=off  i_q_nominal_value=1  i_q_nominal_unit=A  torque_specify=off  torque_priority=None  torque=0 N*m  torque_nominal_specify=off  torque_nominal_value=1  torque_nominal_unit=N*m  angular_velocity_specify=off  angular_velocity_priority=High  angular_velocity=0 rpm  angular_velocity_nominal_specify=off  angular_velocity_nominal_value=1  angular_velocity_nominal_unit=rpm  angular_position_specify=off  angular_position_priority=High  angular_position=0 deg  angular_position_nominal_specify=off  angular_position_nominal_value=1  angular_position_nominal_unit=deg  alpha=0.00393 % Parameter not set 1/K  alpha_flux=-0.001 % Parameter not set 1/K  Tmeas=298.15 % Parameter not set K  stator_thermal_mass=100 % Parameter not set J/K  rotor_thermal_mass=200 % Parameter not set J/K  Rm_percent_rotor=90  Rd_percent_rotor=30  temperatureA_specify=off  temperatureA_priority=High  temperatureA=25 degC  temperatureA_nominal_specify=off  temperatureA_nominal_value=1  temperatureA_nominal_unit=degC  temperatureB_specify=off  temperatureB_priority=High  temperatureB=25 degC  temperatureB_nominal_specify=off  temperatureB_nominal_value=1  temperatureB_nominal_unit=degC  temperatureC_specify=off  temperatureC_priority=High  temperatureC=25 degC  temperatureC_nominal_specify=off  temperatureC_nominal_value=1  temperatureC_nominal_unit=degC  temperatureR_specify=off  temperatureR_priority=High  temperatureR=25 degC  temperatureR_nominal_specify=off  temperatureR_nominal_value=1  temperatureR_nominal_unit=degC
      settings: AttributesFormatString=Maxon:ECXTORQUE_22XL_48  InternalSimscapePortConfiguration="{\"Bottom\":[],\"Left\":[{\"id\":\"N\",\"label\":\"~\",\"type\":\"foundation.electrical.three_phase\"}],\"Right\":[{\"id\":\"R\",\"label\":\"R\",\"type\":\"foundation.mechanical.rotational.rotational\"},{\"id\":\"C\",\"label\":\"C\",\"type\":\"foundation.mechanical.rotational.rotational\"}],\"Top\":[]}"
  Current_Sensor : ee_lib/Sensors & Transducers/Current Sensor (Three-Phase)
  Electrical Reference1 : fl_lib/Electrical/Electrical Elements/Electrical Reference
  Gmin : fl_lib/Electrical/Electrical Elements/Resistor  R=1e9 Ohm  i_specify=off  i_priority=None  i=0 A  i_nominal_specify=off  i_nominal_value=1  i_nominal_unit=A  v_specify=off  v_priority=None  v=0 V  v_nominal_specify=off  v_nominal_value=1  v_nominal_unit=V
  Ideal_Rotational_Mot ion_Sensor : fl_lib/Mechanical/Mechanical Sensors/Ideal Rotational Motion Sensor  reference=foundation.enum.MeasurementReference.difference  acceleration_port=false  velocity_port=true  position_port=true  wrap_angle=simscape.enum.onoff.off  offset=BLDC.RotorPositionInit rad
  Ideal_Torque_Sensor : fl_lib/Mechanical/Mechanical Sensors/Ideal Torque Sensor
  Line Voltage Sensor (Three-Phase) : ee_lib/Sensors & Transducers/Line Voltage Sensor (Three-Phase)
  Measurements : Subsystem
  Mechanical Rotational Reference2 : fl_lib/Mechanical/Rotational Elements/Mechanical Rotational Reference
  PS-Simulink Converter : nesl_utility/PS-Simulink Converter  PhysicalDomain=network_engine_domain  SubClassName=ps_output  LeftPortType=input  RightPortType=output  PseudoPeriodic=off  Frequencies=[]  VectorFormat=inherit  Unit=inherit  AffineConversion=off
  Permanent_Magnet_Synchronous_Motor1 : ee_lib/Electromechanical/Permanent Magnet/PMSM  Commented=on  port_option=ee.enum.threePhasePort.composite  winding_type=ee.enum.statorconnection.wye  machine_param=ee.enum.pmsm.parameterization.constant  nPolePairs=pmsm.PolePairs  pmflux_param=1  pm_flux_linkage=pmsm.FluxLinkage Wb  torque_constant=0.18 N*m/A  back_emf_constant=0.18 V/(rad/s)  stator_param=1  Ld=pmsm.InductanceLd H  Lq=pmsm.InductanceLq H  idVec=[-200, 0, 200] A  iqVec=[-200, 0, 200] A  LdMatrix=0.0002 * ones(3, 3) H  LqMatrix=0.0002 * ones(3, 3) H  PmMatrix=0.1 * ones(3, 3) Wb  ktMatrix=0.18 * ones(3, 3) N*m/A  keMatrix=0.18 * ones(3, 3) V*s/rad  L0=pmsm.InductanceL0 H  Ls=0.0002 H  Lm=0 H  Ms=0 H  Rs=pmsm.StatorPhaseResistance Ohm  zero_sequence=ee.enum.park.zerosequence.include  axes_param=2  loss_param=ee.enum.ironloss.none  losses_oc=[0, 0, 0] W  losses_sc=[0, 0, 0] W  f_losses=60 Hz  Isc_losses=95 A  J=0 kg*m^2  lam=0 N*m/(rad/s)  i_d_specify=off  i_d_priority=None  i_d=0 A  i_d_nominal_specify=off  i_d_nominal_value=1  i_d_nominal_unit=A  i_q_specify=off  i_q_priority=None  i_q=0 A  i_q_nominal_specify=off  i_q_nominal_value=1  i_q_nominal_unit=A  torque_specify=off  torque_priority=None  torque=0 N*m  torque_nominal_specify=off  torque_nominal_value=1  torque_nominal_unit=N*m  angular_velocity_specify=on  angular_velocity_priority=None  angular_velocity=0 rpm  angular_velocity_nominal_specify=off  angular_velocity_nominal_value=1  angular_velocity_nominal_unit=rpm  angular_position_specify=on  angular_position_priority=High  angular_position=pmsm.RotorPositionInit rad  angular_position_nominal_specify=off  angular_position_nominal_value=1  angular_position_nominal_unit=deg  alpha=3.93e-3 1/K  alpha_flux=-0.001 1/K  Tmeas=298.15 K  stator_thermal_mass=100 J/K  rotor_thermal_mass=200 J/K  Rm_percent_rotor=90  Rd_percent_rotor=30  temperatureA_specify=off  temperatureA_priority=High  temperatureA=25 degC  temperatureA_nominal_specify=off  temperatureA_nominal_value=1  temperatureA_nominal_unit=degC  temperatureB_specify=off  temperatureB_priority=High  temperatureB=25 degC  temperatureB_nominal_specify=off  temperatureB_nominal_value=1  temperatureB_nominal_unit=degC  temperatureC_specify=off  temperatureC_priority=High  temperatureC=25 degC  temperatureC_nominal_specify=off  temperatureC_nominal_value=1  temperatureC_nominal_unit=degC  temperatureR_specify=off  temperatureR_priority=High  temperatureR=25 degC  temperatureR_nominal_specify=off  temperatureR_nominal_value=1  temperatureR_nominal_unit=degC
      settings: InternalSimscapePortConfiguration="{\"Bottom\":[],\"Left\":[{\"id\":\"N\",\"label\":\"~\",\"type\":\"foundation.electrical.three_phase\"},{\"id\":\"n\",\"label\":\"n\",\"type\":\"foundation.electrical.electrical\"}],\"Right\":[{\"id\":\"R\",\"label\":\"R\",\"type\":\"foundation.mechanical.rotational.rotational\"},{\"id\":\"C\",\"label\":\"C\",\"type\":\"foundation.mechanical.rotational.rotational\"}],\"Top\":[]}"
  Phase_Splitter : ee_lib/Connectors & References/Phase Splitter
  Rotational_Friction : fl_lib/Mechanical/Rotational Elements/Rotational Friction  brkwy_trq=BLDC.BreakawayFrictionTorque N*m  brkwy_vel=0.060623 rad/s  Col_trq=BLDC.CoulombFrictionTorque N*m  visc_coef=BLDC.ViscousFrictionCoefficient N*m/(rad/s)  w_specify=on  w_priority=Low  w=BLDC.RotorVelocityInit rpm  w_nominal_specify=off  w_nominal_value=1  w_nominal_unit=rad/s  t_specify=off  t_priority=None  t=0 N*m  t_nominal_specify=off  t_nominal_value=1  t_nominal_unit=N*m
  Rotor_Inertia : fl_lib/Mechanical/Rotational Elements/Inertia  inertia=BLDC.Inertia kg*m^2  num_ports=foundation.enum.numPorts2.one  w_specify=on  w_priority=Low  w=BLDC.RotorVelocityInit rpm  w_nominal_specify=off  w_nominal_value=1  w_nominal_unit=rad/s  t_specify=off  t_priority=None  t=0 N*m  t_nominal_specify=off  t_nominal_value=1  t_nominal_unit=N*m
  A : PMIOPort  Side=Left
  B : PMIOPort  Port=2  Side=Left
  C : PMIOPort  Port=3  Side=Left
  R : PMIOPort  Port=4  Side=Right
  M : Outport  VectorParamsAs1DForOutWhenUnconnected=off
  tag scope: abc_output=global
  wires:
  Measurements/1(M) -> M/1
  PS-Simulink Converter/1 -> [abc_output]
  connections:
  Measurements/LConn4 -- Ideal_Rotational_Mot ion_Sensor/RConn2
  Measurements/LConn3 -- Ideal_Rotational_Mot ion_Sensor/RConn3
  Measurements/LConn2 -- Ideal_Torque_Sensor/RConn2
  BLDC/LConn1 -- Current_Sensor/RConn2
  C/RConn1 -- Phase_Splitter/RConn3
  B/RConn1 -- Phase_Splitter/RConn2
  A/RConn1 -- Phase_Splitter/RConn1
  Gmin/RConn1 -- BLDC/LConn2
  Mechanical Rotational Reference2/LConn1 -- Rotational_Friction/RConn1 -- Ideal_Rotational_Mot ion_Sensor/RConn1 -- BLDC/RConn2
  Phase_Splitter/LConn1 -- Current_Sensor/LConn1 -- Line Voltage Sensor (Three-Phase)/LConn1
  Current_Sensor/RConn1 -- Measurements/LConn1
  Electrical Reference1/LConn1 -- Gmin/LConn1
  BLDC/RConn1 -- Ideal_Torque_Sensor/LConn1
  Rotor_Inertia/LConn1 -- Ideal_Rotational_Mot ion_Sensor/LConn1 -- Rotational_Friction/LConn1 -- R/RConn1 -- Ideal_Torque_Sensor/RConn1
  PS-Simulink Converter/LConn1 -- Line Voltage Sensor (Three-Phase)/RConn1

== system BLDC_simulator/Motor_And_Load/Disc_Load ==
  note: Disc Load
  Inertia : fl_lib/Mechanical/Rotational Elements/Inertia  inertia=disc.Inertia kg*m^2  num_ports=foundation.enum.numPorts2.one  w_specify=on  w_priority=High  w=BLDC.RotorVelocityInit rad/s  w_nominal_specify=off  w_nominal_value=1  w_nominal_unit=rad/s  t_specify=off  t_priority=High  t=0 N*m  t_nominal_specify=off  t_nominal_value=1  t_nominal_unit=N*m
      settings: AttributesFormatString=|
      | ---------------------------
      | Inertia = %<inertia>
  R : PMIOPort  Side=Right
  connections:
  Inertia/LConn1 -- R/RConn1

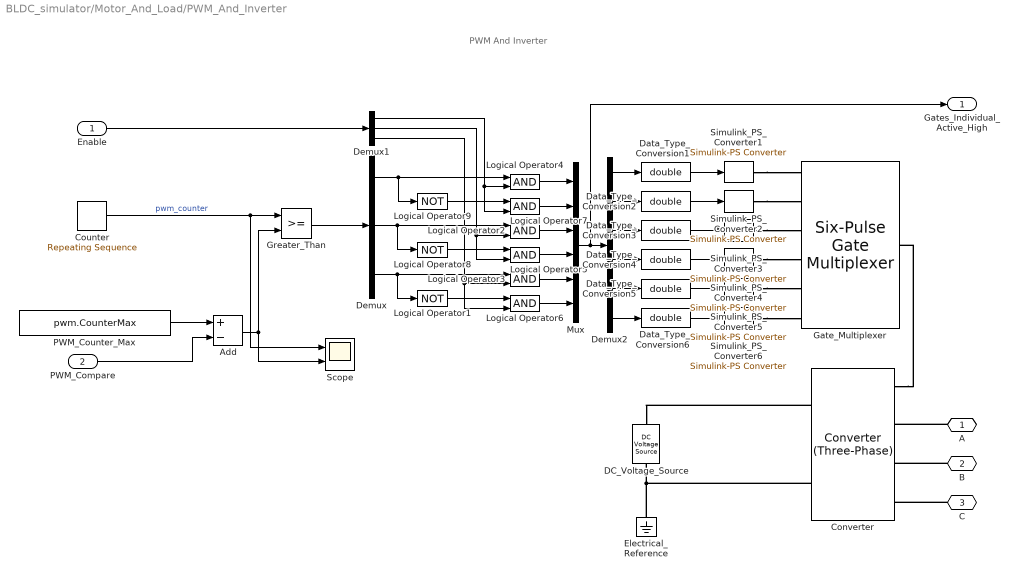
== system BLDC_simulator/Motor_And_Load/PWM_And_Inverter ==
  note: PWM And Inverter
  Enable : Inport
  PWM_Compare : Inport  Port=2
  Add : Sum  Inputs=+-  OutDataTypeStr=Inherit: Same as first input
  Converter : ee_lib/Semiconductors & Converters/Converters/Converter (Three-Phase)  port_option=ee.enum.threePhasePort.expanded  fidelity_option=ee.enum.converters.fidelity.detailed  device_type=2  K=0  Vf=0.8 V  Ron=0.001 Ohm  Rds=0.001 Ohm  Goff=1e-6 1/Ohm  Vgt=1 V  Vgt_off=-1 V  Ih=1 A  Vth=0.5 V  diode_param=1  diode_Vf=0.8 V  diode_Ron=0.001 Ohm  diode_Goff=1e-5 1/Ohm  diode_C=50 nF  diode_iRM=-235 A  diode_iF=300 A  diode_idot=-50 A/us  diode_trr_param=1  diode_trr_factor=3  diode_trr=15 us  diode_Qrr=1.5e+3 s*uA  snubber_type=0  Cs=1e-7 F  Rs=0.1 Ohm
      settings: InternalSimscapePortConfiguration="{\"Bottom\":[],\"Left\":[{\"id\":\"G\",\"label\":\"G\",\"type\":\"foundation.electrical.twelve_phase\"},{\"id\":\"a\",\"label\":\"a\",\"type\":\"foundation.electrical.electrical\"},{\"id\":\"b\",\"label\":\"b\",\"type\":\"foundation.electrical.electrical\"},{\"id\":\"c\",\"label\":\"c\",\"type\":\"foundation.electrical.electrical\"}],\"Right\":[{\"id\":\"p\",\"label\":\"+\",\"type\":\"foundation.electrical.electrical\"},{\"id\":\"n\",\"label\":\"-\",\"type\":\"foundation.electrical.electrical\"}],\"Top\":[]}"
  Counter : simulink/Sources/Repeating Sequence  rep_seq_t=pwm.Period * [0 0.5 1]  rep_seq_y=pwm.CounterMax * [0 1 0]
      settings: AttributesFormatString=|
      | ---------------------------------------
      | Time = %<rep_seq_t>
      | Values = %<rep_seq_y>
  DC_Voltage_Source : fl_lib/Electrical/Electrical Sources/DC Voltage Source  v0=inverter.BusVoltage V
      settings: AttributesFormatString=|
      | ------------------------------------
      | V = %<v0>
  Data_Type_Conversion{1..6} (6 alike) : DataTypeConversion  OutDataTypeStr=double  SaturateOnIntegerOverflow=off  RndMeth=Floor
  Demux : Demux  Outputs=3
  Demux1 : Demux  Outputs=3
  Demux2 : Demux  Outputs=6
  Electrical_Reference : fl_lib/Electrical/Electrical Elements/Electrical Reference
  Gate_Multiplexer : ee_lib/Semiconductors & Converters/Converters/Six-Pulse Gate Multiplexer  port_option=ee.enum.controlport.ps
  Greater_Than : RelationalOperator  OutDataTypeStr=boolean  InputSameDT=off
  Logical Operator1 : Logic  Operator=NOT  IconShape=distinctive  AllPortsSameDT=off  OutDataTypeStr=boolean
  Logical Operator{2..7} (6 alike) : Logic  IconShape=distinctive  AllPortsSameDT=off  OutDataTypeStr=boolean
  Logical Operator8 : Logic  Operator=NOT  IconShape=distinctive  AllPortsSameDT=off  OutDataTypeStr=boolean
  Logical Operator9 : Logic  Operator=NOT  IconShape=distinctive  AllPortsSameDT=off  OutDataTypeStr=boolean
  Mux : Mux  Inputs=6
  PWM_Counter_Max : Constant  Value=pwm.CounterMax  OutDataTypeStr=uint16
  Scope : Scope  NumInputPorts=2
  Simulink_PS_Converter{1..6} (6 alike) : nesl_utility/Simulink-PS Converter  PhysicalDomain=network_engine_domain  SubClassName=ps_input  LeftPortType=input  RightPortType=output  PseudoPeriodic=off  Frequencies=[]  NoiseDistribution=none  NoiseParameters=[]  Unit=1  AffineConversion=off  FilteringAndDerivatives=zero  SimscapeFilterOrder=1  InputFilterTimeConstant=0.001  UdotUserProvided=1
  A : PMIOPort  Side=Right
  B : PMIOPort  Port=2  Side=Right
  C : PMIOPort  Port=3  Side=Right
  Gates_Individual_Active_High : Outport  VectorParamsAs1DForOutWhenUnconnected=off
  wires:
  Data_Type_Conversion6/1 -> Simulink_PS_Converter6/1
  Data_Type_Conversion5/1 -> Simulink_PS_Converter5/1
  Data_Type_Conversion4/1 -> Simulink_PS_Converter4/1
  Data_Type_Conversion3/1 -> Simulink_PS_Converter3/1
  Data_Type_Conversion2/1 -> Simulink_PS_Converter2/1
  Data_Type_Conversion1/1 -> Simulink_PS_Converter1/1
  Demux2/1 -> Data_Type_Conversion1/1
  Demux2/2 -> Data_Type_Conversion2/1
  Demux2/3 -> Data_Type_Conversion3/1
  Demux2/4 -> Data_Type_Conversion4/1
  Demux2/5 -> Data_Type_Conversion5/1
  Demux2/6 -> Data_Type_Conversion6/1
  Mux/1 -> Demux2/1, Gates_Individual_Active_High/1
  Counter/1 -> Scope/1, Greater_Than/1  "pwm_counter"
  Demux/2 -> Logical Operator2/1, Logical Operator8/1
  Logical Operator1/1 -> Logical Operator6/1
  Logical Operator3/1 -> Mux/5
  Demux/1 -> Logical Operator9/1, Logical Operator4/1
  Logical Operator5/1 -> Mux/4
  Logical Operator6/1 -> Mux/6
  Demux1/1 -> Logical Operator4/2, Logical Operator7/2
  Demux1/3 -> Logical Operator6/2, Logical Operator3/2
  Logical Operator9/1 -> Logical Operator7/1
  Demux1/2 -> Logical Operator5/2, Logical Operator2/2
  Logical Operator8/1 -> Logical Operator5/1
  Logical Operator7/1 -> Mux/2
  Logical Operator4/1 -> Mux/1
  Demux/3 -> Logical Operator3/1, Logical Operator1/1
  Logical Operator2/1 -> Mux/3
  Enable/1 -> Demux1/1
  Greater_Than/1 -> Demux/1
  PWM_Compare/1 -> Add/2
  PWM_Counter_Max/1 -> Add/1
  Add/1 -> Greater_Than/2, Scope/2
  connections:
  Simulink_PS_Converter2/RConn1 -- Gate_Multiplexer/LConn2
  Simulink_PS_Converter4/RConn1 -- Gate_Multiplexer/LConn4
  Simulink_PS_Converter6/RConn1 -- Gate_Multiplexer/LConn6
  Converter/LConn1 -- Gate_Multiplexer/RConn1
  C/RConn1 -- Converter/LConn4
  Simulink_PS_Converter1/RConn1 -- Gate_Multiplexer/LConn1
  Simulink_PS_Converter5/RConn1 -- Gate_Multiplexer/LConn5
  Simulink_PS_Converter3/RConn1 -- Gate_Multiplexer/LConn3
  B/RConn1 -- Converter/LConn3
  A/RConn1 -- Converter/LConn2
  Converter/RConn1 -- DC_Voltage_Source/LConn1
  Converter/RConn2 -- DC_Voltage_Source/RConn1 -- Electrical_Reference/LConn1

== system BLDC_simulator/Motor_And_Load/Torque_Load ==
  note: Torque Load
  T : Inport
  Ideal_Torque_Source : fl_lib/Mechanical/Mechanical Sources/Ideal Torque Source
  Mechanical_Rotational_Reference : fl_lib/Mechanical/Rotational Elements/Mechanical Rotational Reference
  Simulink_PS_Converter : nesl_utility/Simulink-PS Converter  PhysicalDomain=network_engine_domain  SubClassName=ps_input  LeftPortType=input  RightPortType=output  PseudoPeriodic=off  Frequencies=[]  NoiseDistribution=none  NoiseParameters=[]  Unit=N*m  AffineConversion=off  FilteringAndDerivatives=zero  SimscapeFilterOrder=1  InputFilterTimeConstant=.001  UdotUserProvided=1
  R : PMIOPort  Side=Right
  wires:
  T/1 -> Simulink_PS_Converter/1  "loadTorque"
  connections:
  Ideal_Torque_Source/LConn1 -- R/RConn1
  Simulink_PS_Converter/RConn1 -- Ideal_Torque_Source/RConn1
  Mechanical_Rotational_Reference/LConn1 -- Ideal_Torque_Source/RConn2
